simulink model "SolarCar"  (R2025b)
settings: Solver=VariableStepAuto  StartTime=0.0  StopTime=10.0  RelTol=1e-3
undefined symbols (not defined in the file): Line
(part 1 of 2)
settings Model: Creator=nhtyn  LastModifiedBy=nhtyn

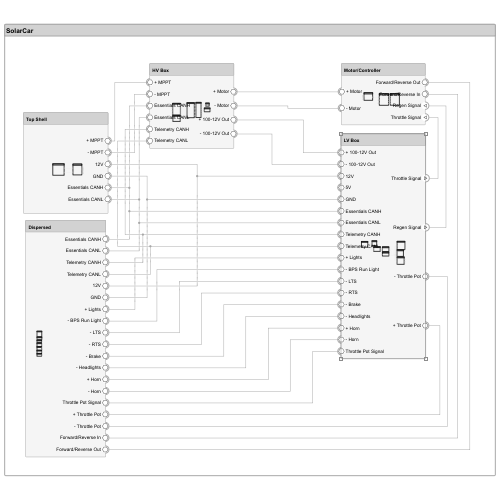
[thumbnail: Simulink's stored preview of the top-level diagram]
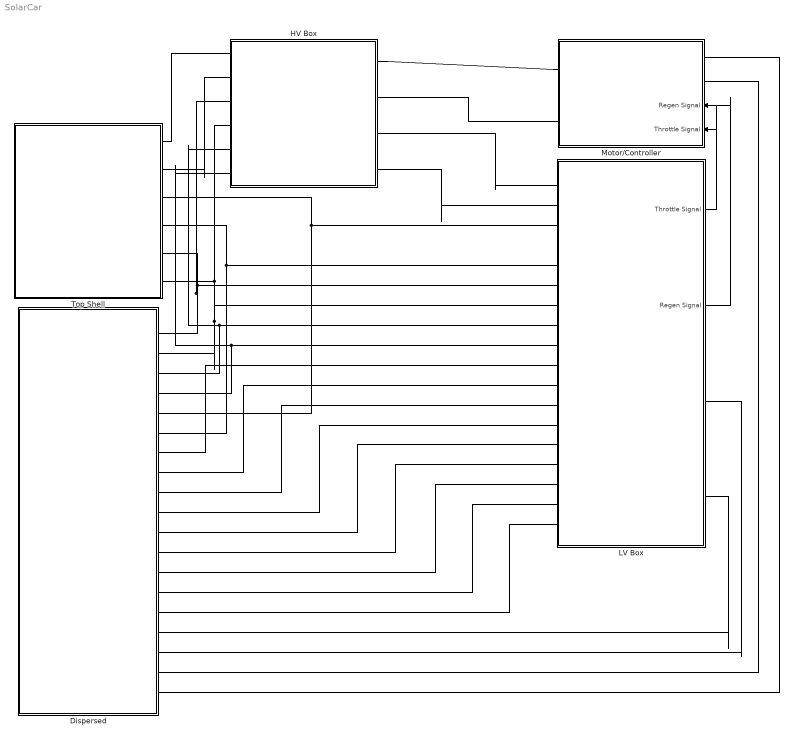
== system SolarCar ==
  Dispersed : Subsystem
      settings: PortSchema="{\"entries\":[{\"content\":{\"headerSize\":26,\"margin\":15,\"minimumSpacing\":25,\"sides\":[{\"content\":{},\"type\":\"ConnectorPlacement.EquallySpacedRectSide\",\"uuid\":\"bc47d88e-4b1b-4064-ab24-769f2538e68d\"},{\"content\":{\"connectorIds\":[\"RConn1\",\"RConn2\",\"RConn3\",\"RConn4\",\"RConn5\",\"RConn6\",\"RConn7\",\"RConn8\",\"RConn9\",\"RConn10\",\"RConn11\",\"RConn12\",\"RConn13\",\"RConn14\",\"RConn15\",\"RConn16\",\"RConn17\",\"RConn18\",\"RConn19\"],\"side\":\"RIGHT\"},\"type\":\"ConnectorPlacement.EquallySpacedRectSide\",\"uuid\":\"fdd62b94-80f2-4d2e-a8f3-223633e3a920\"},{\"content\":{\"side\":\"TOP\"},\"type\":\"ConnectorPlacement.EquallySpacedRectSide\",\"uuid\":\"e8df0b32-bf38-452a-bef9-69ccd7b44596\"}]},\"type\":\"ConnectorPlacement.EquallySpacedConnector\",\"uuid\":\"127e4cb3-ba30-47ff-b0d0-2c5b6f0f1031\"}],\"packageUris\":[\"http://schema.mathworks.com/mf0/Connector/R2020b\"],\"version\":\"1.0\"}"
  HV Box : Subsystem
      settings: PortSchema="{\"entries\":[{\"content\":{\"headerSize\":26,\"margin\":15,\"minimumSpacing\":25,\"sides\":[{\"content\":{\"connectorIds\":[\"RConn5\",\"RConn6\",\"LConn1\",\"LConn2\",\"LConn3\",\"LConn4\"]},\"type\":\"ConnectorPlacement.EquallySpacedRectSide\",\"uuid\":\"c92e0290-dc73-43e5-9f21-68f158b061d1\"},{\"content\":{\"connectorIds\":[\"RConn1\",\"RConn2\",\"RConn3\",\"RConn4\"],\"side\":\"RIGHT\"},\"type\":\"ConnectorPlacement.EquallySpacedRectSide\",\"uuid\":\"be8eb41d-7a66-441b-b503-1306464e1273\"},{\"content\":{\"side\":\"TOP\"},\"type\":\"ConnectorPlacement.EquallySpacedRectSide\",\"uuid\":\"34016d46-a56f-490a-9c85-32531a59f6cc\"}]},\"type\":\"ConnectorPlacement.EquallySpacedConnector\",\"uuid\":\"21576b4b-d4ce-437a-96c9-76a257c64a5e\"}],\"packageUris\":[\"http://schema.mathworks.com/mf0/Connector/R2020b\"],\"version\":\"1.0\"}"
  LV Box : Subsystem
      settings: PortSchema="{\"entries\":[{\"content\":{\"headerSize\":26,\"margin\":15,\"minimumSpacing\":25,\"sides\":[{\"content\":{\"connectorIds\":[\"LConn1\",\"LConn2\",\"LConn3\",\"LConn4\",\"LConn5\",\"LConn6\",\"LConn7\",\"LConn8\",\"LConn9\",\"LConn10\",\"LConn11\",\"LConn12\",\"LConn13\",\"LConn14\",\"LConn15\",\"LConn16\",\"LConn17\",\"LConn18\"]},\"type\":\"ConnectorPlacement.EquallySpacedRectSide\",\"uuid\":\"c92e0290-dc73-43e5-9f21-68f158b061d1\"},{\"content\":{\"connectorIds\":[\"Out1\",\"Out2\",\"RConn2\",\"RConn1\"],\"side\":\"RIGHT\"},\"type\":\"ConnectorPlacement.EquallySpacedRectSide\",\"uuid\":\"be8eb41d-7a66-441b-b503-1306464e1273\"},{\"content\":{\"side\":\"TOP\"},\"type\":\"ConnectorPlacement.EquallySpacedRectSide\",\"uuid\":\"34016d46-a56f-490a-9c85-32531a59f6cc\"}]},\"type\":\"ConnectorPlacement.EquallySpacedConnector\",\"uuid\":\"21576b4b-d4ce-437a-96c9-76a257c64a5e\"}],\"packageUris\":[\"http://schema.mathworks.com/mf0/Connector/R2020b\"],\"version\":\"1.0\"}"
  Motor/Controller : Subsystem
      settings: PortSchema="{\"entries\":[{\"content\":{\"headerSize\":26,\"margin\":15,\"minimumSpacing\":25,\"sides\":[{\"content\":{\"connectorIds\":[\"LConn1\",\"LConn2\"]},\"type\":\"ConnectorPlacement.EquallySpacedRectSide\",\"uuid\":\"c92e0290-dc73-43e5-9f21-68f158b061d1\"},{\"content\":{\"connectorIds\":[\"RConn1\",\"RConn2\",\"In2\",\"In1\"],\"side\":\"RIGHT\"},\"type\":\"ConnectorPlacement.EquallySpacedRectSide\",\"uuid\":\"be8eb41d-7a66-441b-b503-1306464e1273\"},{\"content\":{\"side\":\"TOP\"},\"type\":\"ConnectorPlacement.EquallySpacedRectSide\",\"uuid\":\"34016d46-a56f-490a-9c85-32531a59f6cc\"}]},\"type\":\"ConnectorPlacement.EquallySpacedConnector\",\"uuid\":\"21576b4b-d4ce-437a-96c9-76a257c64a5e\"}],\"packageUris\":[\"http://schema.mathworks.com/mf0/Connector/R2020b\"],\"version\":\"1.0\"}"
  Top Shell : Subsystem
      settings: PortSchema="{\"entries\":[{\"content\":{\"headerSize\":26,\"margin\":15,\"minimumSpacing\":25,\"sides\":[{\"content\":{},\"type\":\"ConnectorPlacement.EquallySpacedRectSide\",\"uuid\":\"c92e0290-dc73-43e5-9f21-68f158b061d1\"},{\"content\":{\"connectorIds\":[\"RConn1\",\"RConn2\",\"RConn3\",\"RConn4\",\"RConn5\",\"RConn6\"],\"side\":\"RIGHT\"},\"type\":\"ConnectorPlacement.EquallySpacedRectSide\",\"uuid\":\"be8eb41d-7a66-441b-b503-1306464e1273\"},{\"content\":{\"side\":\"TOP\"},\"type\":\"ConnectorPlacement.EquallySpacedRectSide\",\"uuid\":\"34016d46-a56f-490a-9c85-32531a59f6cc\"}]},\"type\":\"ConnectorPlacement.EquallySpacedConnector\",\"uuid\":\"21576b4b-d4ce-437a-96c9-76a257c64a5e\"}],\"packageUris\":[\"http://schema.mathworks.com/mf0/Connector/R2020b\"],\"version\":\"1.0\"}"
  wires:
  LV Box/1(Throttle Signal) -> Motor/Controller/1(Throttle Signal)
  LV Box/2(Regen Signal) -> Motor/Controller/2(Regen Signal)
  connections:
  Dispersed/RConn1 -- HV Box/LConn1 -- Top Shell/RConn5 -- LV Box/LConn6
  Top Shell/RConn6 -- HV Box/LConn2 -- Dispersed/RConn2 -- LV Box/LConn7
  HV Box/RConn1 -- Motor/Controller/LConn1
  HV Box/RConn2 -- Motor/Controller/LConn2
  HV Box/RConn5 -- Top Shell/RConn1
  HV Box/RConn6 -- Top Shell/RConn2
  HV Box/RConn3 -- LV Box/LConn1
  HV Box/RConn4 -- LV Box/LConn2
  LV Box/LConn8 -- Dispersed/RConn3 -- HV Box/LConn3
  LV Box/LConn9 -- Dispersed/RConn4 -- HV Box/LConn4
  LV Box/LConn10 -- Dispersed/RConn7
  LV Box/LConn11 -- Dispersed/RConn8
  LV Box/LConn12 -- Dispersed/RConn9
  LV Box/LConn13 -- Dispersed/RConn10
  LV Box/LConn14 -- Dispersed/RConn11
  LV Box/LConn15 -- Dispersed/RConn12
  Dispersed/RConn13 -- LV Box/LConn16
  Dispersed/RConn14 -- LV Box/LConn17
  LV Box/LConn18 -- Dispersed/RConn15
  LV Box/RConn1 -- Dispersed/RConn16
  LV Box/RConn2 -- Dispersed/RConn17
  LV Box/LConn3 -- Top Shell/RConn3 -- Dispersed/RConn5
  LV Box/LConn5 -- Dispersed/RConn6 -- Top Shell/RConn4
  Dispersed/RConn18 -- Motor/Controller/RConn2
  Dispersed/RConn19 -- Motor/Controller/RConn1

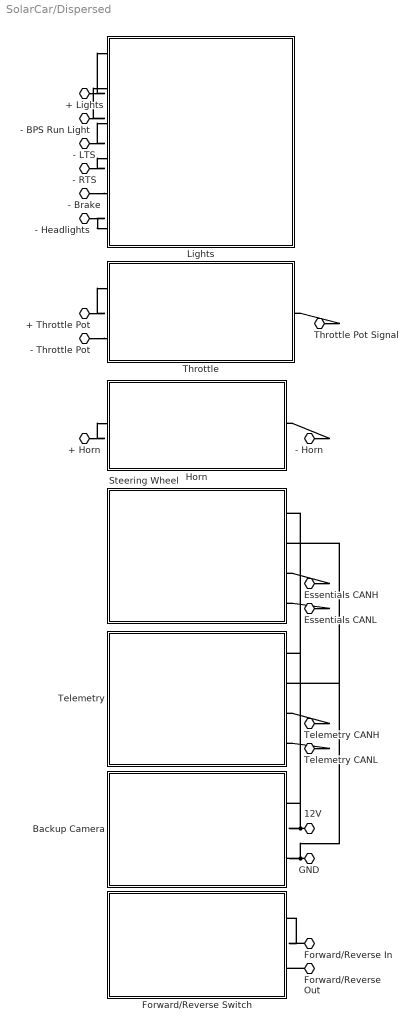
== system SolarCar/Dispersed ==
  Backup Camera : Subsystem
      settings: PortSchema="{\"entries\":[{\"content\":{\"headerSize\":26,\"margin\":15,\"minimumSpacing\":25,\"sides\":[{\"content\":{},\"type\":\"ConnectorPlacement.EquallySpacedRectSide\",\"uuid\":\"16c5a28a-8204-43c6-ae1e-ca56bf00262c\"},{\"content\":{\"connectorIds\":[\"RConn1\",\"RConn2\"],\"side\":\"RIGHT\"},\"type\":\"ConnectorPlacement.EquallySpacedRectSide\",\"uuid\":\"d50f7b79-0d90-4c13-9b04-ddd7ba1c0b17\"},{\"content\":{\"side\":\"TOP\"},\"type\":\"ConnectorPlacement.EquallySpacedRectSide\",\"uuid\":\"232c283e-7372-4332-942a-1b4711a4445f\"}]},\"type\":\"ConnectorPlacement.EquallySpacedConnector\",\"uuid\":\"38533706-c242-4f43-b565-c99062dd3fc1\"}],\"packageUris\":[\"http://schema.mathworks.com/mf0/Connector/R2020b\"],\"version\":\"1.0\"}"
  Forward/Reverse Switch : Subsystem
      settings: PortSchema="{\"entries\":[{\"content\":{\"headerSize\":26,\"margin\":15,\"minimumSpacing\":25,\"sides\":[{\"content\":{},\"type\":\"ConnectorPlacement.EquallySpacedRectSide\",\"uuid\":\"16c5a28a-8204-43c6-ae1e-ca56bf00262c\"},{\"content\":{\"connectorIds\":[\"RConn1\",\"RConn2\"],\"side\":\"RIGHT\"},\"type\":\"ConnectorPlacement.EquallySpacedRectSide\",\"uuid\":\"d50f7b79-0d90-4c13-9b04-ddd7ba1c0b17\"},{\"content\":{\"side\":\"TOP\"},\"type\":\"ConnectorPlacement.EquallySpacedRectSide\",\"uuid\":\"232c283e-7372-4332-942a-1b4711a4445f\"}]},\"type\":\"ConnectorPlacement.EquallySpacedConnector\",\"uuid\":\"38533706-c242-4f43-b565-c99062dd3fc1\"}],\"packageUris\":[\"http://schema.mathworks.com/mf0/Connector/R2020b\"],\"version\":\"1.0\"}"
  Horn : Subsystem
      settings: PortSchema="{\"entries\":[{\"content\":{\"headerSize\":26,\"margin\":15,\"minimumSpacing\":25,\"sides\":[{\"content\":{\"connectorIds\":[\"LConn1\"]},\"type\":\"ConnectorPlacement.EquallySpacedRectSide\",\"uuid\":\"16c5a28a-8204-43c6-ae1e-ca56bf00262c\"},{\"content\":{\"connectorIds\":[\"RConn1\"],\"side\":\"RIGHT\"},\"type\":\"ConnectorPlacement.EquallySpacedRectSide\",\"uuid\":\"d50f7b79-0d90-4c13-9b04-ddd7ba1c0b17\"},{\"content\":{\"side\":\"TOP\"},\"type\":\"ConnectorPlacement.EquallySpacedRectSide\",\"uuid\":\"232c283e-7372-4332-942a-1b4711a4445f\"}]},\"type\":\"ConnectorPlacement.EquallySpacedConnector\",\"uuid\":\"38533706-c242-4f43-b565-c99062dd3fc1\"}],\"packageUris\":[\"http://schema.mathworks.com/mf0/Connector/R2020b\"],\"version\":\"1.0\"}"
  Lights : Subsystem
      settings: PortSchema="{\"entries\":[{\"content\":{\"headerSize\":26,\"margin\":15,\"minimumSpacing\":25,\"sides\":[{\"content\":{\"connectorIds\":[\"LConn1\",\"LConn2\",\"LConn3\",\"LConn4\",\"LConn5\",\"LConn6\"]},\"type\":\"ConnectorPlacement.EquallySpacedRectSide\",\"uuid\":\"16c5a28a-8204-43c6-ae1e-ca56bf00262c\"},{\"content\":{\"side\":\"RIGHT\"},\"type\":\"ConnectorPlacement.EquallySpacedRectSide\",\"uuid\":\"d50f7b79-0d90-4c13-9b04-ddd7ba1c0b17\"},{\"content\":{\"side\":\"TOP\"},\"type\":\"ConnectorPlacement.EquallySpacedRectSide\",\"uuid\":\"232c283e-7372-4332-942a-1b4711a4445f\"}]},\"type\":\"ConnectorPlacement.EquallySpacedConnector\",\"uuid\":\"38533706-c242-4f43-b565-c99062dd3fc1\"}],\"packageUris\":[\"http://schema.mathworks.com/mf0/Connector/R2020b\"],\"version\":\"1.0\"}"
  Steering Wheel : Subsystem
      settings: PortSchema="{\"entries\":[{\"content\":{\"headerSize\":26,\"margin\":15,\"minimumSpacing\":25,\"sides\":[{\"content\":{},\"type\":\"ConnectorPlacement.EquallySpacedRectSide\",\"uuid\":\"bc47d88e-4b1b-4064-ab24-769f2538e68d\"},{\"content\":{\"connectorIds\":[\"RConn1\",\"RConn2\",\"RConn3\",\"RConn4\"],\"side\":\"RIGHT\"},\"type\":\"ConnectorPlacement.EquallySpacedRectSide\",\"uuid\":\"fdd62b94-80f2-4d2e-a8f3-223633e3a920\"},{\"content\":{\"side\":\"TOP\"},\"type\":\"ConnectorPlacement.EquallySpacedRectSide\",\"uuid\":\"e8df0b32-bf38-452a-bef9-69ccd7b44596\"}]},\"type\":\"ConnectorPlacement.EquallySpacedConnector\",\"uuid\":\"127e4cb3-ba30-47ff-b0d0-2c5b6f0f1031\"}],\"packageUris\":[\"http://schema.mathworks.com/mf0/Connector/R2020b\"],\"version\":\"1.0\"}"
  Telemetry : Subsystem
      settings: PortSchema="{\"entries\":[{\"content\":{\"headerSize\":26,\"margin\":15,\"minimumSpacing\":25,\"sides\":[{\"content\":{},\"type\":\"ConnectorPlacement.EquallySpacedRectSide\",\"uuid\":\"bc47d88e-4b1b-4064-ab24-769f2538e68d\"},{\"content\":{\"connectorIds\":[\"RConn1\",\"RConn2\",\"RConn3\",\"RConn4\"],\"side\":\"RIGHT\"},\"type\":\"ConnectorPlacement.EquallySpacedRectSide\",\"uuid\":\"fdd62b94-80f2-4d2e-a8f3-223633e3a920\"},{\"content\":{\"side\":\"TOP\"},\"type\":\"ConnectorPlacement.EquallySpacedRectSide\",\"uuid\":\"e8df0b32-bf38-452a-bef9-69ccd7b44596\"}]},\"type\":\"ConnectorPlacement.EquallySpacedConnector\",\"uuid\":\"127e4cb3-ba30-47ff-b0d0-2c5b6f0f1031\"}],\"packageUris\":[\"http://schema.mathworks.com/mf0/Connector/R2020b\"],\"version\":\"1.0\"}"
  Throttle : Subsystem
      settings: PortSchema="{\"entries\":[{\"content\":{\"headerSize\":26,\"margin\":15,\"minimumSpacing\":25,\"sides\":[{\"content\":{\"connectorIds\":[\"LConn1\",\"LConn2\"]},\"type\":\"ConnectorPlacement.EquallySpacedRectSide\",\"uuid\":\"16c5a28a-8204-43c6-ae1e-ca56bf00262c\"},{\"content\":{\"connectorIds\":[\"RConn1\"],\"side\":\"RIGHT\"},\"type\":\"ConnectorPlacement.EquallySpacedRectSide\",\"uuid\":\"d50f7b79-0d90-4c13-9b04-ddd7ba1c0b17\"},{\"content\":{\"side\":\"TOP\"},\"type\":\"ConnectorPlacement.EquallySpacedRectSide\",\"uuid\":\"232c283e-7372-4332-942a-1b4711a4445f\"}]},\"type\":\"ConnectorPlacement.EquallySpacedConnector\",\"uuid\":\"38533706-c242-4f43-b565-c99062dd3fc1\"}],\"packageUris\":[\"http://schema.mathworks.com/mf0/Connector/R2020b\"],\"version\":\"1.0\"}"
  Essentials CANH : PMIOPort  Side=Right
  Essentials CANL : PMIOPort  Port=2  Side=Right
  Telemetry CANH : PMIOPort  Port=3  Side=Right
  Telemetry CANL : PMIOPort  Port=4  Side=Right
  12V : PMIOPort  Port=5  Side=Right
  GND : PMIOPort  Port=6  Side=Right
  + Lights : PMIOPort  Port=7  Side=Right
  - BPS Run Light : PMIOPort  Port=8  Side=Right
  - LTS : PMIOPort  Port=9  Side=Right
  - RTS : PMIOPort  Port=10  Side=Right
  - Brake : PMIOPort  Port=11  Side=Right
  - Headlights : PMIOPort  Port=12  Side=Right
  + Horn : PMIOPort  Port=13  Side=Right
  - Horn : PMIOPort  Port=14  Side=Right
  Throttle Pot Signal : PMIOPort  Port=15  Side=Right
  + Throttle Pot : PMIOPort  Port=16  Side=Right
  - Throttle Pot : PMIOPort  Port=17  Side=Right
  Forward/Reverse In : PMIOPort  Port=18  Side=Right
  Forward/Reverse Out : PMIOPort  Port=19  Side=Right
  connections:
  Essentials CANH/RConn1 -- Steering Wheel/RConn3
  Essentials CANL/RConn1 -- Steering Wheel/RConn4
  + Lights/RConn1 -- Lights/LConn1
  - BPS Run Light/RConn1 -- Lights/LConn2
  - LTS/RConn1 -- Lights/LConn3
  - RTS/RConn1 -- Lights/LConn4
  - Brake/RConn1 -- Lights/LConn5
  - Headlights/RConn1 -- Lights/LConn6
  + Horn/RConn1 -- Horn/LConn1
  - Horn/RConn1 -- Horn/RConn1
  + Throttle Pot/RConn1 -- Throttle/LConn1
  - Throttle Pot/RConn1 -- Throttle/LConn2
  Throttle Pot Signal/RConn1 -- Throttle/RConn1
  Forward/Reverse In/RConn1 -- Forward/Reverse Switch/RConn1
  Forward/Reverse Out/RConn1 -- Forward/Reverse Switch/RConn2
  12V/RConn1 -- Telemetry/RConn1 -- Steering Wheel/RConn1 -- Backup Camera/RConn1
  GND/RConn1 -- Telemetry/RConn2 -- Steering Wheel/RConn2 -- Backup Camera/RConn2
  Telemetry CANH/RConn1 -- Telemetry/RConn3
  Telemetry CANL/RConn1 -- Telemetry/RConn4

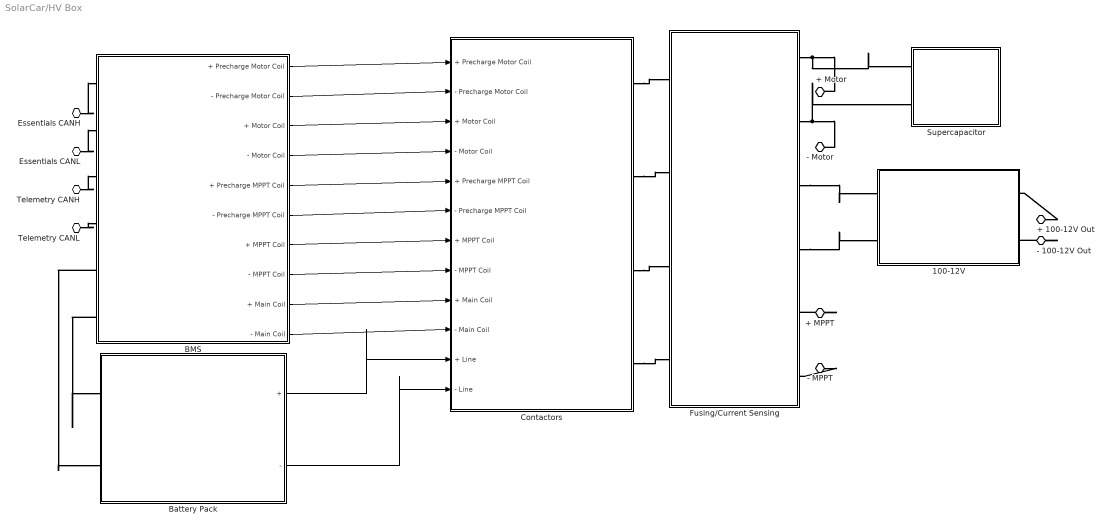
== system SolarCar/HV Box ==
  100-12V : Subsystem
      settings: PortSchema="{\"entries\":[{\"content\":{\"headerSize\":26,\"margin\":15,\"minimumSpacing\":25,\"sides\":[{\"content\":{\"connectorIds\":[\"LConn1\",\"LConn2\"]},\"type\":\"ConnectorPlacement.EquallySpacedRectSide\",\"uuid\":\"c92e0290-dc73-43e5-9f21-68f158b061d1\"},{\"content\":{\"connectorIds\":[\"RConn1\",\"RConn2\"],\"side\":\"RIGHT\"},\"type\":\"ConnectorPlacement.EquallySpacedRectSide\",\"uuid\":\"be8eb41d-7a66-441b-b503-1306464e1273\"},{\"content\":{\"side\":\"TOP\"},\"type\":\"ConnectorPlacement.EquallySpacedRectSide\",\"uuid\":\"34016d46-a56f-490a-9c85-32531a59f6cc\"}]},\"type\":\"ConnectorPlacement.EquallySpacedConnector\",\"uuid\":\"21576b4b-d4ce-437a-96c9-76a257c64a5e\"}],\"packageUris\":[\"http://schema.mathworks.com/mf0/Connector/R2020b\"],\"version\":\"1.0\"}"
  BMS : Subsystem
      settings: PortSchema="{\"entries\":[{\"content\":{\"headerSize\":26,\"margin\":15,\"minimumSpacing\":25,\"sides\":[{\"content\":{\"connectorIds\":[\"LConn1\",\"LConn2\",\"LConn3\",\"LConn4\",\"LConn5\",\"LConn6\"]},\"type\":\"ConnectorPlacement.EquallySpacedRectSide\",\"uuid\":\"c92e0290-dc73-43e5-9f21-68f158b061d1\"},{\"content\":{\"connectorIds\":[\"Out1\",\"Out2\",\"Out3\",\"Out4\",\"Out5\",\"Out6\",\"Out7\",\"Out8\",\"Out9\",\"Out10\"],\"side\":\"RIGHT\"},\"type\":\"ConnectorPlacement.EquallySpacedRectSide\",\"uuid\":\"be8eb41d-7a66-441b-b503-1306464e1273\"},{\"content\":{\"side\":\"TOP\"},\"type\":\"ConnectorPlacement.EquallySpacedRectSide\",\"uuid\":\"34016d46-a56f-490a-9c85-32531a59f6cc\"},{\"content\":{\"side\":\"BOTTOM\"},\"type\":\"ConnectorPlacement.EquallySpacedRectSide\",\"uuid\":\"f63c834d-6003-4ec6-8d44-6b3bc1c3f4f7\"}]},\"type\":\"ConnectorPlacement.EquallySpacedConnector\",\"uuid\":\"21576b4b-d4ce-437a-96c9-76a257c64a5e\"}],\"packageUris\":[\"http://schema.mathworks.com/mf0/Connector/R2020b\"],\"version\":\"1.0\"}"
  Battery Pack : Subsystem
      settings: PortSchema="{\"entries\":[{\"content\":{\"headerSize\":26,\"margin\":15,\"minimumSpacing\":25,\"sides\":[{\"content\":{\"connectorIds\":[\"LConn1\",\"LConn2\"]},\"type\":\"ConnectorPlacement.EquallySpacedRectSide\",\"uuid\":\"c92e0290-dc73-43e5-9f21-68f158b061d1\"},{\"content\":{\"connectorIds\":[\"Out1\",\"Out2\"],\"side\":\"RIGHT\"},\"type\":\"ConnectorPlacement.EquallySpacedRectSide\",\"uuid\":\"be8eb41d-7a66-441b-b503-1306464e1273\"},{\"content\":{\"side\":\"TOP\"},\"type\":\"ConnectorPlacement.EquallySpacedRectSide\",\"uuid\":\"34016d46-a56f-490a-9c85-32531a59f6cc\"}]},\"type\":\"ConnectorPlacement.EquallySpacedConnector\",\"uuid\":\"21576b4b-d4ce-437a-96c9-76a257c64a5e\"}],\"packageUris\":[\"http://schema.mathworks.com/mf0/Connector/R2020b\"],\"version\":\"1.0\"}"
  Contactors : Subsystem
      settings: PortSchema="{\"entries\":[{\"content\":{\"headerSize\":26,\"margin\":15,\"minimumSpacing\":25,\"sides\":[{\"content\":{\"connectorIds\":[\"In1\",\"In2\",\"In3\",\"In4\",\"In5\",\"In6\",\"In7\",\"In8\",\"In9\",\"In10\",\"In11\",\"In12\"]},\"type\":\"ConnectorPlacement.EquallySpacedRectSide\",\"uuid\":\"a524e60d-b40a-408b-8bd2-a27c555355ac\"},{\"content\":{\"connectorIds\":[\"RConn1\",\"RConn3\",\"RConn2\",\"RConn4\"],\"side\":\"RIGHT\"},\"type\":\"ConnectorPlacement.EquallySpacedRectSide\",\"uuid\":\"88e19f78-eac2-4161-9d7e-9c49ae9957fc\"},{\"content\":{\"side\":\"TOP\"},\"type\":\"ConnectorPlacement.EquallySpacedRectSide\",\"uuid\":\"b9255ea4-184a-49ec-9d1c-02386d46c5b2\"}]},\"type\":\"ConnectorPlacement.EquallySpacedConnector\",\"uuid\":\"32913e94-0913-4a3c-90e8-81be48841784\"}],\"packageUris\":[\"http://schema.mathworks.com/mf0/Connector/R2020b\"],\"version\":\"1.0\"}"
  Fusing/Current Sensing : Subsystem
      settings: PortSchema="{\"entries\":[{\"content\":{\"headerSize\":26,\"margin\":15,\"minimumSpacing\":25,\"sides\":[{\"content\":{\"connectorIds\":[\"LConn1\",\"LConn4\",\"LConn2\",\"LConn3\"]},\"type\":\"ConnectorPlacement.EquallySpacedRectSide\",\"uuid\":\"16c5a28a-8204-43c6-ae1e-ca56bf00262c\"},{\"content\":{\"connectorIds\":[\"RConn1\",\"RConn3\",\"RConn2\",\"RConn4\",\"RConn5\",\"RConn6\"],\"side\":\"RIGHT\"},\"type\":\"ConnectorPlacement.EquallySpacedRectSide\",\"uuid\":\"d50f7b79-0d90-4c13-9b04-ddd7ba1c0b17\"},{\"content\":{\"side\":\"TOP\"},\"type\":\"ConnectorPlacement.EquallySpacedRectSide\",\"uuid\":\"232c283e-7372-4332-942a-1b4711a4445f\"}]},\"type\":\"ConnectorPlacement.EquallySpacedConnector\",\"uuid\":\"38533706-c242-4f43-b565-c99062dd3fc1\"}],\"packageUris\":[\"http://schema.mathworks.com/mf0/Connector/R2020b\"],\"version\":\"1.0\"}"
  Supercapacitor : Subsystem
      settings: PortSchema="{\"entries\":[{\"content\":{\"headerSize\":26,\"margin\":15,\"minimumSpacing\":25,\"sides\":[{\"content\":{\"connectorIds\":[\"LConn1\",\"LConn2\"]},\"type\":\"ConnectorPlacement.EquallySpacedRectSide\",\"uuid\":\"7f164fa2-9272-4d7a-9d1b-73fbad559026\"},{\"content\":{\"side\":\"RIGHT\"},\"type\":\"ConnectorPlacement.EquallySpacedRectSide\",\"uuid\":\"4e5c1bb6-197d-43aa-a880-a6796570230e\"},{\"content\":{\"side\":\"TOP\"},\"type\":\"ConnectorPlacement.EquallySpacedRectSide\",\"uuid\":\"a6abaace-1014-4cef-9d43-479b6863617c\"}]},\"type\":\"ConnectorPlacement.EquallySpacedConnector\",\"uuid\":\"97f01c5b-0fe0-4837-90bc-01d73eb3d078\"}],\"packageUris\":[\"http://schema.mathworks.com/mf0/Connector/R2020b\"],\"version\":\"1.0\"}"
  + Motor : PMIOPort  Side=Right
  - Motor : PMIOPort  Port=2  Side=Right
  + 100-12V Out : PMIOPort  Port=3  Side=Right
  - 100-12V Out : PMIOPort  Port=4  Side=Right
  + MPPT : PMIOPort  Port=5  Side=Right
  - MPPT : PMIOPort  Port=6  Side=Right
  Essentials CANH : PMIOPort  Port=7  Side=Left
  Essentials CANL : PMIOPort  Port=8  Side=Left
  Telemetry CANH : PMIOPort  Port=9  Side=Left
  Telemetry CANL : PMIOPort  Port=10  Side=Left
  wires:
  BMS/1(+ Precharge Motor Coil) -> Contactors/1(+ Precharge Motor Coil)
  BMS/2(- Precharge Motor Coil) -> Contactors/2(- Precharge Motor Coil)
  BMS/3(+ Motor Coil) -> Contactors/3(+ Motor Coil)
  Battery Pack/1(+) -> Contactors/11(+ Line)
  Battery Pack/2(-) -> Contactors/12(- Line)
  BMS/4(- Motor Coil) -> Contactors/4(- Motor Coil)
  BMS/5(+ Precharge MPPT Coil) -> Contactors/5(+ Precharge MPPT Coil)
  BMS/6(- Precharge MPPT Coil) -> Contactors/6(- Precharge MPPT Coil)
  BMS/7(+ MPPT Coil) -> Contactors/7(+ MPPT Coil)
  BMS/8(- MPPT Coil) -> Contactors/8(- MPPT Coil)
  BMS/9(+ Main Coil) -> Contactors/9(+ Main Coil)
  BMS/10(- Main Coil) -> Contactors/10(- Main Coil)
  connections:
  Contactors/RConn4 -- Fusing/Current Sensing/LConn3
  Contactors/RConn3 -- Fusing/Current Sensing/LConn4
  Contactors/RConn1 -- Fusing/Current Sensing/LConn1
  Contactors/RConn2 -- Fusing/Current Sensing/LConn2
  Fusing/Current Sensing/RConn2 -- 100-12V/LConn1
  Fusing/Current Sensing/RConn4 -- 100-12V/LConn2
  Fusing/Current Sensing/RConn1 -- Supercapacitor/LConn1 -- + Motor/RConn1
  Fusing/Current Sensing/RConn3 -- Supercapacitor/LConn2 -- - Motor/RConn1
  - MPPT/RConn1 -- Fusing/Current Sensing/RConn6
  + MPPT/RConn1 -- Fusing/Current Sensing/RConn5
  + 100-12V Out/RConn1 -- 100-12V/RConn1
  - 100-12V Out/RConn1 -- 100-12V/RConn2
  Essentials CANH/RConn1 -- BMS/LConn1
  Essentials CANL/RConn1 -- BMS/LConn2
  Telemetry CANH/RConn1 -- BMS/LConn3
  Telemetry CANL/RConn1 -- BMS/LConn4
  BMS/LConn5 -- Battery Pack/LConn2
  BMS/LConn6 -- Battery Pack/LConn1

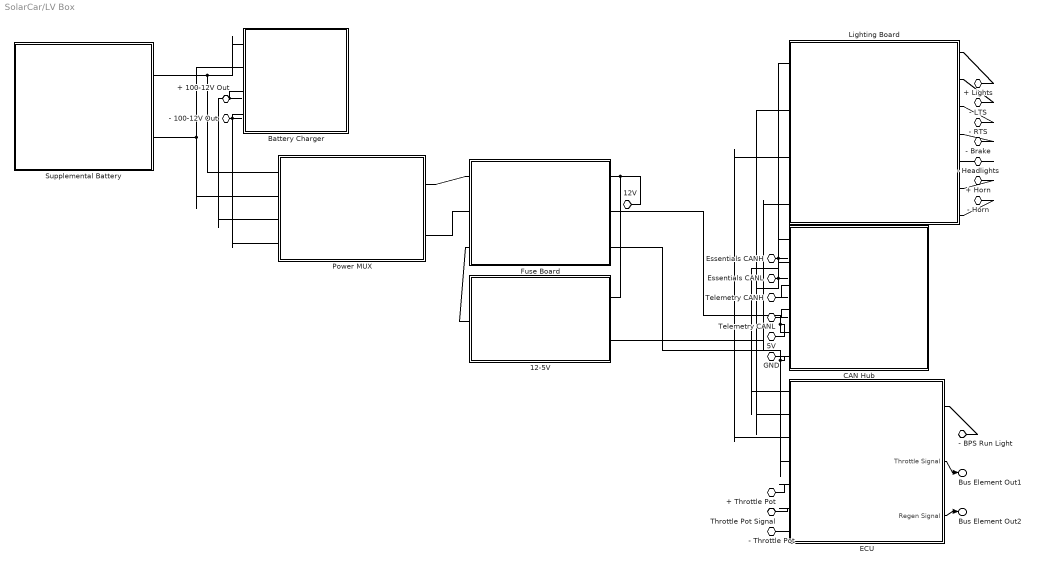
== system SolarCar/LV Box ==
  12-5V : Subsystem
      settings: PortSchema="{\"entries\":[{\"content\":{\"headerSize\":26,\"margin\":15,\"minimumSpacing\":25,\"sides\":[{\"content\":{\"connectorIds\":[\"RConn1\"]},\"type\":\"ConnectorPlacement.EquallySpacedRectSide\",\"uuid\":\"e398aa85-cf01-454b-8c65-40a3b68188cb\"},{\"content\":{\"connectorIds\":[\"LConn1\",\"LConn2\"],\"side\":\"RIGHT\"},\"type\":\"ConnectorPlacement.EquallySpacedRectSide\",\"uuid\":\"9e40fc98-7fa4-4457-a2a2-72d8b3bd46fd\"},{\"content\":{\"side\":\"TOP\"},\"type\":\"ConnectorPlacement.EquallySpacedRectSide\",\"uuid\":\"c0cef17d-c612-441a-9462-c940c3f96980\"}]},\"type\":\"ConnectorPlacement.EquallySpacedConnector\",\"uuid\":\"0ce439f7-0020-43e2-bdb3-8e0f3c386e01\"}],\"packageUris\":[\"http://schema.mathworks.com/mf0/Connector/R2020b\"],\"version\":\"1.0\"}"
  Battery Charger : Subsystem
      settings: PortSchema="{\"entries\":[{\"content\":{\"headerSize\":26,\"margin\":15,\"minimumSpacing\":25,\"sides\":[{\"content\":{\"connectorIds\":[\"LConn1\",\"LConn2\",\"RConn1\",\"RConn2\"]},\"type\":\"ConnectorPlacement.EquallySpacedRectSide\",\"uuid\":\"7f164fa2-9272-4d7a-9d1b-73fbad559026\"},{\"content\":{\"side\":\"RIGHT\"},\"type\":\"ConnectorPlacement.EquallySpacedRectSide\",\"uuid\":\"4e5c1bb6-197d-43aa-a880-a6796570230e\"},{\"content\":{\"side\":\"TOP\"},\"type\":\"ConnectorPlacement.EquallySpacedRectSide\",\"uuid\":\"a6abaace-1014-4cef-9d43-479b6863617c\"}]},\"type\":\"ConnectorPlacement.EquallySpacedConnector\",\"uuid\":\"97f01c5b-0fe0-4837-90bc-01d73eb3d078\"}],\"packageUris\":[\"http://schema.mathworks.com/mf0/Connector/R2020b\"],\"version\":\"1.0\"}"
  CAN Hub : Subsystem
      settings: PortSchema="{\"entries\":[{\"content\":{\"headerSize\":26,\"margin\":15,\"minimumSpacing\":25,\"sides\":[{\"content\":{\"connectorIds\":[\"LConn1\",\"LConn2\",\"LConn3\",\"LConn4\",\"LConn5\",\"LConn6\"]},\"type\":\"ConnectorPlacement.EquallySpacedRectSide\",\"uuid\":\"16c5a28a-8204-43c6-ae1e-ca56bf00262c\"},{\"content\":{\"side\":\"RIGHT\"},\"type\":\"ConnectorPlacement.EquallySpacedRectSide\",\"uuid\":\"d50f7b79-0d90-4c13-9b04-ddd7ba1c0b17\"},{\"content\":{\"side\":\"TOP\"},\"type\":\"ConnectorPlacement.EquallySpacedRectSide\",\"uuid\":\"232c283e-7372-4332-942a-1b4711a4445f\"}]},\"type\":\"ConnectorPlacement.EquallySpacedConnector\",\"uuid\":\"38533706-c242-4f43-b565-c99062dd3fc1\"}],\"packageUris\":[\"http://schema.mathworks.com/mf0/Connector/R2020b\"],\"version\":\"1.0\"}"
  ECU : Subsystem
      settings: PortSchema="{\"entries\":[{\"content\":{\"headerSize\":26,\"margin\":15,\"minimumSpacing\":25,\"sides\":[{\"content\":{\"connectorIds\":[\"LConn1\",\"LConn2\",\"LConn3\",\"LConn4\",\"LConn5\",\"LConn6\",\"LConn7\"]},\"type\":\"ConnectorPlacement.EquallySpacedRectSide\",\"uuid\":\"c92e0290-dc73-43e5-9f21-68f158b061d1\"},{\"content\":{\"connectorIds\":[\"RConn1\",\"Out1\",\"Out2\"],\"side\":\"RIGHT\"},\"type\":\"ConnectorPlacement.EquallySpacedRectSide\",\"uuid\":\"be8eb41d-7a66-441b-b503-1306464e1273\"},{\"content\":{\"side\":\"TOP\"},\"type\":\"ConnectorPlacement.EquallySpacedRectSide\",\"uuid\":\"34016d46-a56f-490a-9c85-32531a59f6cc\"}]},\"type\":\"ConnectorPlacement.EquallySpacedConnector\",\"uuid\":\"21576b4b-d4ce-437a-96c9-76a257c64a5e\"}],\"packageUris\":[\"http://schema.mathworks.com/mf0/Connector/R2020b\"],\"version\":\"1.0\"}"
  Fuse Board : Subsystem
      settings: PortSchema="{\"entries\":[{\"content\":{\"headerSize\":26,\"margin\":15,\"minimumSpacing\":25,\"sides\":[{\"content\":{\"connectorIds\":[\"LConn1\",\"LConn2\",\"LConn3\"]},\"type\":\"ConnectorPlacement.EquallySpacedRectSide\",\"uuid\":\"c92e0290-dc73-43e5-9f21-68f158b061d1\"},{\"content\":{\"connectorIds\":[\"RConn1\",\"RConn2\",\"RConn3\"],\"side\":\"RIGHT\"},\"type\":\"ConnectorPlacement.EquallySpacedRectSide\",\"uuid\":\"be8eb41d-7a66-441b-b503-1306464e1273\"},{\"content\":{\"side\":\"TOP\"},\"type\":\"ConnectorPlacement.EquallySpacedRectSide\",\"uuid\":\"34016d46-a56f-490a-9c85-32531a59f6cc\"}]},\"type\":\"ConnectorPlacement.EquallySpacedConnector\",\"uuid\":\"21576b4b-d4ce-437a-96c9-76a257c64a5e\"}],\"packageUris\":[\"http://schema.mathworks.com/mf0/Connector/R2020b\"],\"version\":\"1.0\"}"
  Lighting Board : Subsystem
      settings: PortSchema="{\"entries\":[{\"content\":{\"headerSize\":26,\"margin\":15,\"minimumSpacing\":25,\"sides\":[{\"content\":{\"connectorIds\":[\"LConn1\",\"LConn2\",\"LConn3\",\"LConn4\"]},\"type\":\"ConnectorPlacement.EquallySpacedRectSide\",\"uuid\":\"c92e0290-dc73-43e5-9f21-68f158b061d1\"},{\"content\":{\"connectorIds\":[\"RConn2\",\"RConn3\",\"RConn1\",\"RConn4\",\"RConn5\",\"RConn6\",\"RConn7\"],\"side\":\"RIGHT\"},\"type\":\"ConnectorPlacement.EquallySpacedRectSide\",\"uuid\":\"be8eb41d-7a66-441b-b503-1306464e1273\"},{\"content\":{\"side\":\"TOP\"},\"type\":\"ConnectorPlacement.EquallySpacedRectSide\",\"uuid\":\"34016d46-a56f-490a-9c85-32531a59f6cc\"},{\"content\":{\"side\":\"BOTTOM\"},\"type\":\"ConnectorPlacement.EquallySpacedRectSide\",\"uuid\":\"089da668-218a-4509-a90e-e522bf51239f\"}]},\"type\":\"ConnectorPlacement.EquallySpacedConnector\",\"uuid\":\"21576b4b-d4ce-437a-96c9-76a257c64a5e\"}],\"packageUris\":[\"http://schema.mathworks.com/mf0/Connector/R2020b\"],\"version\":\"1.0\"}"
  Power MUX : Subsystem
      settings: PortSchema="{\"entries\":[{\"content\":{\"headerSize\":26,\"margin\":15,\"minimumSpacing\":25,\"sides\":[{\"content\":{\"connectorIds\":[\"LConn1\",\"LConn2\",\"LConn3\",\"RConn3\"]},\"type\":\"ConnectorPlacement.EquallySpacedRectSide\",\"uuid\":\"c92e0290-dc73-43e5-9f21-68f158b061d1\"},{\"content\":{\"connectorIds\":[\"RConn1\",\"RConn2\"],\"side\":\"RIGHT\"},\"type\":\"ConnectorPlacement.EquallySpacedRectSide\",\"uuid\":\"be8eb41d-7a66-441b-b503-1306464e1273\"},{\"content\":{\"side\":\"TOP\"},\"type\":\"ConnectorPlacement.EquallySpacedRectSide\",\"uuid\":\"34016d46-a56f-490a-9c85-32531a59f6cc\"},{\"content\":{\"side\":\"BOTTOM\"},\"type\":\"ConnectorPlacement.EquallySpacedRectSide\",\"uuid\":\"c5320d22-5298-4b0f-919e-298988f1412c\"}]},\"type\":\"ConnectorPlacement.EquallySpacedConnector\",\"uuid\":\"21576b4b-d4ce-437a-96c9-76a257c64a5e\"}],\"packageUris\":[\"http://schema.mathworks.com/mf0/Connector/R2020b\"],\"version\":\"1.0\"}"
  Supplemental Battery : Subsystem
      settings: PortSchema="{\"entries\":[{\"content\":{\"headerSize\":26,\"margin\":15,\"minimumSpacing\":25,\"sides\":[{\"content\":{},\"type\":\"ConnectorPlacement.EquallySpacedRectSide\",\"uuid\":\"c92e0290-dc73-43e5-9f21-68f158b061d1\"},{\"content\":{\"connectorIds\":[\"RConn1\",\"RConn2\"],\"side\":\"RIGHT\"},\"type\":\"ConnectorPlacement.EquallySpacedRectSide\",\"uuid\":\"be8eb41d-7a66-441b-b503-1306464e1273\"},{\"content\":{\"side\":\"TOP\"},\"type\":\"ConnectorPlacement.EquallySpacedRectSide\",\"uuid\":\"34016d46-a56f-490a-9c85-32531a59f6cc\"}]},\"type\":\"ConnectorPlacement.EquallySpacedConnector\",\"uuid\":\"21576b4b-d4ce-437a-96c9-76a257c64a5e\"}],\"packageUris\":[\"http://schema.mathworks.com/mf0/Connector/R2020b\"],\"version\":\"1.0\"}"
  + 100-12V Out : PMIOPort  Side=Left
  - 100-12V Out : PMIOPort  Port=2  Side=Left
  12V : PMIOPort  Port=3  Side=Left
  5V : PMIOPort  Port=4  Side=Left
  GND : PMIOPort  Port=5  Side=Left
  Essentials CANH : PMIOPort  Port=6  Side=Left
  Essentials CANL : PMIOPort  Port=7  Side=Left
  Telemetry CANH : PMIOPort  Port=8  Side=Left
  Telemetry CANL : PMIOPort  Port=9  Side=Left
  + Lights : PMIOPort  Port=10  Side=Left
  - BPS Run Light : PMIOPort  Port=11  Side=Left
  - LTS : PMIOPort  Port=12  Side=Left
  - RTS : PMIOPort  Port=13  Side=Left
  - Brake : PMIOPort  Port=14  Side=Left
  - Headlights : PMIOPort  Port=15  Side=Left
  + Horn : PMIOPort  Port=16  Side=Left
  - Horn : PMIOPort  Port=17  Side=Left
  + Throttle Pot : PMIOPort  Port=18  Side=Right
  - Throttle Pot : PMIOPort  Port=19  Side=Right
  Throttle Pot Signal : PMIOPort  Port=20  Side=Left
  Bus Element Out1 : Outport  PortName=Throttle Signal
  Bus Element Out2 : Outport  Port=2  PortName=Regen Signal
  wires:
  ECU/1(Throttle Signal) -> Bus Element Out1/1
  ECU/2(Regen Signal) -> Bus Element Out2/1
  connections:
  Essentials CANH/RConn1 -- CAN Hub/LConn1 -- Lighting Board/LConn1 -- ECU/LConn1
  Essentials CANL/RConn1 -- CAN Hub/LConn2 -- Lighting Board/LConn2 -- ECU/LConn2
  + Lights/RConn1 -- Lighting Board/RConn2
  - LTS/RConn1 -- Lighting Board/RConn3
  - RTS/RConn1 -- Lighting Board/RConn1
  - Brake/RConn1 -- Lighting Board/RConn4
  - Headlights/RConn1 -- Lighting Board/RConn5
  Telemetry CANH/RConn1 -- CAN Hub/LConn3
  Telemetry CANL/RConn1 -- CAN Hub/LConn4
  Supplemental Battery/RConn1 -- Battery Charger/LConn1 -- Power MUX/LConn1
  Supplemental Battery/RConn2 -- Battery Charger/LConn2 -- Power MUX/LConn2
  + 100-12V Out/RConn1 -- Battery Charger/RConn1 -- Power MUX/LConn3
  - 100-12V Out/RConn1 -- Battery Charger/RConn2 -- Power MUX/RConn3
  Power MUX/RConn1 -- Fuse Board/LConn1
  Power MUX/RConn2 -- Fuse Board/LConn2
  ECU/LConn5 -- + Throttle Pot/RConn1
  ECU/LConn7 -- - Throttle Pot/RConn1
  ECU/LConn6 -- Throttle Pot Signal/RConn1
  + Horn/RConn1 -- Lighting Board/RConn6
  - Horn/RConn1 -- Lighting Board/RConn7
  - BPS Run Light/RConn1 -- ECU/RConn1
  Fuse Board/RConn3 -- CAN Hub/LConn6 -- ECU/LConn4 -- 12-5V/LConn2 -- Lighting Board/LConn4 -- GND/RConn1
  Fuse Board/RConn1 -- 12V/RConn1 -- 12-5V/LConn1
  12-5V/RConn1 -- Fuse Board/LConn3
  Fuse Board/RConn2 -- ECU/LConn3 -- CAN Hub/LConn5 -- Lighting Board/LConn3 -- 5V/RConn1

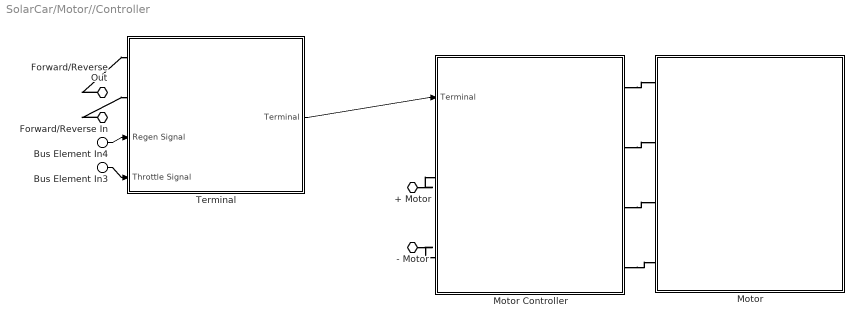
== system SolarCar/Motor//Controller ==
  Bus Element In3 : Inport  PortName=Throttle Signal
  Bus Element In4 : Inport  Port=2  PortName=Regen Signal
  Motor : Subsystem
      settings: PortSchema="{\"entries\":[{\"content\":{\"headerSize\":26,\"margin\":15,\"minimumSpacing\":25,\"sides\":[{\"content\":{\"connectorIds\":[\"LConn1\",\"LConn2\",\"LConn3\",\"LConn4\"]},\"type\":\"ConnectorPlacement.EquallySpacedRectSide\",\"uuid\":\"c92e0290-dc73-43e5-9f21-68f158b061d1\"},{\"content\":{\"side\":\"RIGHT\"},\"type\":\"ConnectorPlacement.EquallySpacedRectSide\",\"uuid\":\"be8eb41d-7a66-441b-b503-1306464e1273\"},{\"content\":{\"side\":\"TOP\"},\"type\":\"ConnectorPlacement.EquallySpacedRectSide\",\"uuid\":\"34016d46-a56f-490a-9c85-32531a59f6cc\"}]},\"type\":\"ConnectorPlacement.EquallySpacedConnector\",\"uuid\":\"21576b4b-d4ce-437a-96c9-76a257c64a5e\"}],\"packageUris\":[\"http://schema.mathworks.com/mf0/Connector/R2020b\"],\"version\":\"1.0\"}"
  Motor Controller : Subsystem
      settings: PortSchema="{\"entries\":[{\"content\":{\"headerSize\":26,\"margin\":15,\"minimumSpacing\":25,\"sides\":[{\"content\":{\"connectorIds\":[\"In1\",\"LConn1\",\"LConn2\"]},\"type\":\"ConnectorPlacement.EquallySpacedRectSide\",\"uuid\":\"c92e0290-dc73-43e5-9f21-68f158b061d1\"},{\"content\":{\"connectorIds\":[\"RConn1\",\"RConn2\",\"RConn3\",\"RConn4\"],\"side\":\"RIGHT\"},\"type\":\"ConnectorPlacement.EquallySpacedRectSide\",\"uuid\":\"be8eb41d-7a66-441b-b503-1306464e1273\"},{\"content\":{\"side\":\"TOP\"},\"type\":\"ConnectorPlacement.EquallySpacedRectSide\",\"uuid\":\"34016d46-a56f-490a-9c85-32531a59f6cc\"}]},\"type\":\"ConnectorPlacement.EquallySpacedConnector\",\"uuid\":\"21576b4b-d4ce-437a-96c9-76a257c64a5e\"}],\"packageUris\":[\"http://schema.mathworks.com/mf0/Connector/R2020b\"],\"version\":\"1.0\"}"
  Terminal : Subsystem
      settings: PortSchema="{\"entries\":[{\"content\":{\"headerSize\":26,\"margin\":15,\"minimumSpacing\":25,\"sides\":[{\"content\":{\"connectorIds\":[\"LConn1\",\"LConn2\",\"In1\",\"In2\"]},\"type\":\"ConnectorPlacement.EquallySpacedRectSide\",\"uuid\":\"16c5a28a-8204-43c6-ae1e-ca56bf00262c\"},{\"content\":{\"connectorIds\":[\"Out1\"],\"side\":\"RIGHT\"},\"type\":\"ConnectorPlacement.EquallySpacedRectSide\",\"uuid\":\"d50f7b79-0d90-4c13-9b04-ddd7ba1c0b17\"},{\"content\":{\"side\":\"TOP\"},\"type\":\"ConnectorPlacement.EquallySpacedRectSide\",\"uuid\":\"232c283e-7372-4332-942a-1b4711a4445f\"}]},\"type\":\"ConnectorPlacement.EquallySpacedConnector\",\"uuid\":\"38533706-c242-4f43-b565-c99062dd3fc1\"}],\"packageUris\":[\"http://schema.mathworks.com/mf0/Connector/R2020b\"],\"version\":\"1.0\"}"
  + Motor : PMIOPort  Side=Left
  - Motor : PMIOPort  Port=2  Side=Left
  Forward/Reverse Out : PMIOPort  Port=3  Side=Right
  Forward/Reverse In : PMIOPort  Port=4  Side=Right
  wires:
  Terminal/1(Terminal) -> Motor Controller/1(Terminal)
  Bus Element In4/1 -> Terminal/1(Regen Signal)
  Bus Element In3/1 -> Terminal/2(Throttle Signal)
  connections:
  + Motor/RConn1 -- Motor Controller/LConn1
  Motor Controller/RConn1 -- Motor/LConn1
  Motor Controller/RConn2 -- Motor/LConn2
  Motor Controller/RConn3 -- Motor/LConn3
  Motor Controller/RConn4 -- Motor/LConn4
  Forward/Reverse Out/RConn1 -- Terminal/LConn1
  Forward/Reverse In/RConn1 -- Terminal/LConn2
  - Motor/RConn1 -- Motor Controller/LConn2

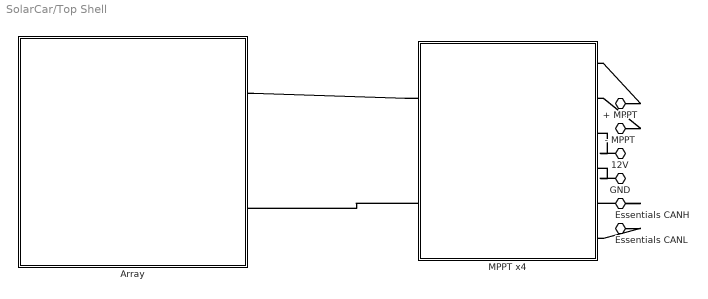
== system SolarCar/Top Shell ==
  Array : Subsystem
      settings: PortSchema="{\"entries\":[{\"content\":{\"headerSize\":26,\"margin\":15,\"minimumSpacing\":25,\"sides\":[{\"content\":{},\"type\":\"ConnectorPlacement.EquallySpacedRectSide\",\"uuid\":\"e398aa85-cf01-454b-8c65-40a3b68188cb\"},{\"content\":{\"connectorIds\":[\"RConn1\",\"RConn2\"],\"side\":\"RIGHT\"},\"type\":\"ConnectorPlacement.EquallySpacedRectSide\",\"uuid\":\"9e40fc98-7fa4-4457-a2a2-72d8b3bd46fd\"},{\"content\":{\"side\":\"TOP\"},\"type\":\"ConnectorPlacement.EquallySpacedRectSide\",\"uuid\":\"c0cef17d-c612-441a-9462-c940c3f96980\"}]},\"type\":\"ConnectorPlacement.EquallySpacedConnector\",\"uuid\":\"0ce439f7-0020-43e2-bdb3-8e0f3c386e01\"}],\"packageUris\":[\"http://schema.mathworks.com/mf0/Connector/R2020b\"],\"version\":\"1.0\"}"
  MPPT x4 : Subsystem
      settings: PortSchema="{\"entries\":[{\"content\":{\"headerSize\":26,\"margin\":15,\"minimumSpacing\":25,\"sides\":[{\"content\":{\"connectorIds\":[\"LConn1\",\"LConn2\"]},\"type\":\"ConnectorPlacement.EquallySpacedRectSide\",\"uuid\":\"e398aa85-cf01-454b-8c65-40a3b68188cb\"},{\"content\":{\"connectorIds\":[\"RConn1\",\"RConn2\",\"RConn3\",\"RConn4\",\"RConn5\",\"RConn6\"],\"side\":\"RIGHT\"},\"type\":\"ConnectorPlacement.EquallySpacedRectSide\",\"uuid\":\"9e40fc98-7fa4-4457-a2a2-72d8b3bd46fd\"},{\"content\":{\"side\":\"TOP\"},\"type\":\"ConnectorPlacement.EquallySpacedRectSide\",\"uuid\":\"c0cef17d-c612-441a-9462-c940c3f96980\"}]},\"type\":\"ConnectorPlacement.EquallySpacedConnector\",\"uuid\":\"0ce439f7-0020-43e2-bdb3-8e0f3c386e01\"}],\"packageUris\":[\"http://schema.mathworks.com/mf0/Connector/R2020b\"],\"version\":\"1.0\"}"
  + MPPT : PMIOPort  Side=Right
  - MPPT : PMIOPort  Port=2  Side=Right
  12V : PMIOPort  Port=3  Side=Right
  GND : PMIOPort  Port=4  Side=Right
  Essentials CANH : PMIOPort  Port=5  Side=Right
  Essentials CANL : PMIOPort  Port=6  Side=Right
  connections:
  Essentials CANH/RConn1 -- MPPT x4/RConn5
  Essentials CANL/RConn1 -- MPPT x4/RConn6
  + MPPT/RConn1 -- MPPT x4/RConn1
  - MPPT/RConn1 -- MPPT x4/RConn2
  MPPT x4/LConn1 -- Array/RConn1
  MPPT x4/LConn2 -- Array/RConn2
  GND/RConn1 -- MPPT x4/RConn4
  12V/RConn1 -- MPPT x4/RConn3

== system SolarCar/Dispersed/Backup Camera ==
  12V : PMIOPort  Side=Right
  GND : PMIOPort  Port=2  Side=Right

== system SolarCar/Dispersed/Forward//Reverse Switch ==
  Forward/Reverse In : PMIOPort  Side=Right
  Forward/Reverse Out : PMIOPort  Port=2  Side=Right

== system SolarCar/Dispersed/Horn ==
  + Horn : PMIOPort  Side=Left
  - Horn : PMIOPort  Port=2  Side=Right

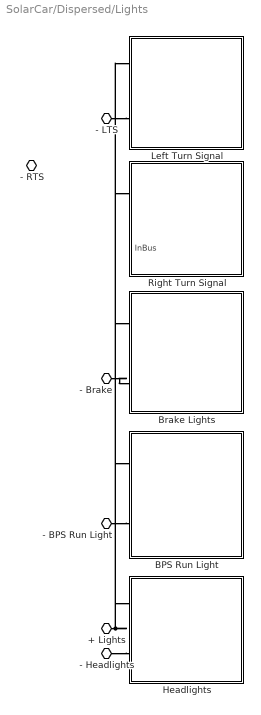
== system SolarCar/Dispersed/Lights ==
  BPS Run Light : Subsystem
      settings: PortSchema="{\"entries\":[{\"content\":{\"headerSize\":26,\"margin\":15,\"minimumSpacing\":25,\"sides\":[{\"content\":{\"connectorIds\":[\"LConn1\",\"LConn2\"]},\"type\":\"ConnectorPlacement.EquallySpacedRectSide\",\"uuid\":\"16c5a28a-8204-43c6-ae1e-ca56bf00262c\"},{\"content\":{\"side\":\"RIGHT\"},\"type\":\"ConnectorPlacement.EquallySpacedRectSide\",\"uuid\":\"d50f7b79-0d90-4c13-9b04-ddd7ba1c0b17\"},{\"content\":{\"side\":\"TOP\"},\"type\":\"ConnectorPlacement.EquallySpacedRectSide\",\"uuid\":\"232c283e-7372-4332-942a-1b4711a4445f\"}]},\"type\":\"ConnectorPlacement.EquallySpacedConnector\",\"uuid\":\"38533706-c242-4f43-b565-c99062dd3fc1\"}],\"packageUris\":[\"http://schema.mathworks.com/mf0/Connector/R2020b\"],\"version\":\"1.0\"}"
  Brake Lights : Subsystem
      settings: PortSchema="{\"entries\":[{\"content\":{\"headerSize\":26,\"margin\":15,\"minimumSpacing\":25,\"sides\":[{\"content\":{\"connectorIds\":[\"LConn1\",\"LConn2\"]},\"type\":\"ConnectorPlacement.EquallySpacedRectSide\",\"uuid\":\"16c5a28a-8204-43c6-ae1e-ca56bf00262c\"},{\"content\":{\"side\":\"RIGHT\"},\"type\":\"ConnectorPlacement.EquallySpacedRectSide\",\"uuid\":\"d50f7b79-0d90-4c13-9b04-ddd7ba1c0b17\"},{\"content\":{\"side\":\"TOP\"},\"type\":\"ConnectorPlacement.EquallySpacedRectSide\",\"uuid\":\"232c283e-7372-4332-942a-1b4711a4445f\"}]},\"type\":\"ConnectorPlacement.EquallySpacedConnector\",\"uuid\":\"38533706-c242-4f43-b565-c99062dd3fc1\"}],\"packageUris\":[\"http://schema.mathworks.com/mf0/Connector/R2020b\"],\"version\":\"1.0\"}"
  Headlights : Subsystem
      settings: PortSchema="{\"entries\":[{\"content\":{\"headerSize\":26,\"margin\":15,\"minimumSpacing\":25,\"sides\":[{\"content\":{\"connectorIds\":[\"LConn1\",\"LConn2\"]},\"type\":\"ConnectorPlacement.EquallySpacedRectSide\",\"uuid\":\"16c5a28a-8204-43c6-ae1e-ca56bf00262c\"},{\"content\":{\"side\":\"RIGHT\"},\"type\":\"ConnectorPlacement.EquallySpacedRectSide\",\"uuid\":\"d50f7b79-0d90-4c13-9b04-ddd7ba1c0b17\"},{\"content\":{\"side\":\"TOP\"},\"type\":\"ConnectorPlacement.EquallySpacedRectSide\",\"uuid\":\"232c283e-7372-4332-942a-1b4711a4445f\"}]},\"type\":\"ConnectorPlacement.EquallySpacedConnector\",\"uuid\":\"38533706-c242-4f43-b565-c99062dd3fc1\"}],\"packageUris\":[\"http://schema.mathworks.com/mf0/Connector/R2020b\"],\"version\":\"1.0\"}"
  Left Turn Signal : Subsystem
      settings: PortSchema="{\"entries\":[{\"content\":{\"headerSize\":26,\"margin\":15,\"minimumSpacing\":25,\"sides\":[{\"content\":{\"connectorIds\":[\"LConn1\",\"LConn2\"]},\"type\":\"ConnectorPlacement.EquallySpacedRectSide\",\"uuid\":\"16c5a28a-8204-43c6-ae1e-ca56bf00262c\"},{\"content\":{\"side\":\"RIGHT\"},\"type\":\"ConnectorPlacement.EquallySpacedRectSide\",\"uuid\":\"d50f7b79-0d90-4c13-9b04-ddd7ba1c0b17\"},{\"content\":{\"side\":\"TOP\"},\"type\":\"ConnectorPlacement.EquallySpacedRectSide\",\"uuid\":\"232c283e-7372-4332-942a-1b4711a4445f\"}]},\"type\":\"ConnectorPlacement.EquallySpacedConnector\",\"uuid\":\"38533706-c242-4f43-b565-c99062dd3fc1\"}],\"packageUris\":[\"http://schema.mathworks.com/mf0/Connector/R2020b\"],\"version\":\"1.0\"}"
  Right Turn Signal : Subsystem
      settings: PortSchema="{\"entries\":[{\"content\":{\"headerSize\":26,\"margin\":15,\"minimumSpacing\":25,\"sides\":[{\"content\":{\"connectorIds\":[\"LConn1\",\"In1\"]},\"type\":\"ConnectorPlacement.EquallySpacedRectSide\",\"uuid\":\"16c5a28a-8204-43c6-ae1e-ca56bf00262c\"},{\"content\":{\"side\":\"RIGHT\"},\"type\":\"ConnectorPlacement.EquallySpacedRectSide\",\"uuid\":\"d50f7b79-0d90-4c13-9b04-ddd7ba1c0b17\"},{\"content\":{\"side\":\"TOP\"},\"type\":\"ConnectorPlacement.EquallySpacedRectSide\",\"uuid\":\"232c283e-7372-4332-942a-1b4711a4445f\"}]},\"type\":\"ConnectorPlacement.EquallySpacedConnector\",\"uuid\":\"38533706-c242-4f43-b565-c99062dd3fc1\"}],\"packageUris\":[\"http://schema.mathworks.com/mf0/Connector/R2020b\"],\"version\":\"1.0\"}"
  + Lights : PMIOPort  Side=Left
  - BPS Run Light : PMIOPort  Port=2  Side=Left
  - LTS : PMIOPort  Port=3  Side=Left
  - RTS : PMIOPort  Port=4  Side=Left
  - Brake : PMIOPort  Port=5  Side=Left
  - Headlights : PMIOPort  Port=6  Side=Left
  wires:
  ? -> Right Turn Signal/1(InBus)
  connections:
  + Lights/RConn1 -- Right Turn Signal/LConn1 -- Left Turn Signal/LConn1 -- Brake Lights/LConn1 -- BPS Run Light/LConn1 -- Headlights/LConn1
  - BPS Run Light/RConn1 -- BPS Run Light/LConn2
  - LTS/RConn1 -- Left Turn Signal/LConn2
  - Brake/RConn1 -- Brake Lights/LConn2
  - Headlights/RConn1 -- Headlights/LConn2

== system SolarCar/Dispersed/Steering Wheel ==
  12V : PMIOPort  Side=Right
  GND : PMIOPort  Port=2  Side=Right
  Essentials CANH : PMIOPort  Port=3  Side=Right
  Essentials CANL : PMIOPort  Port=4  Side=Right

== system SolarCar/Dispersed/Telemetry ==
  12V : PMIOPort  Side=Right
  GND : PMIOPort  Port=2  Side=Right
  Telemetry CANH : PMIOPort  Port=3  Side=Right
  Telemetry CANL : PMIOPort  Port=4  Side=Right

== system SolarCar/Dispersed/Throttle ==
  + Throttle Pot : PMIOPort  Side=Left
  - Throttle Pot : PMIOPort  Port=2  Side=Left
  Throttle Pot Signal : PMIOPort  Port=3  Side=Right

== system SolarCar/HV Box/100-12V ==
  + 100-12V In : PMIOPort  Side=Left
  - 100-12V In : PMIOPort  Port=2  Side=Left
  + 100-12V Out : PMIOPort  Port=3  Side=Right
  - 100-12V Out : PMIOPort  Port=4  Side=Right

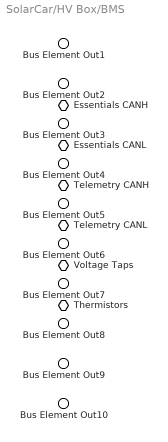
== system SolarCar/HV Box/BMS ==
  Essentials CANH : PMIOPort  Side=Left
  Essentials CANL : PMIOPort  Port=2  Side=Left
  Telemetry CANH : PMIOPort  Port=3  Side=Left
  Telemetry CANL : PMIOPort  Port=4  Side=Left
  Voltage Taps : PMIOPort  Port=5  Side=Left
  Thermistors : PMIOPort  Port=6  Side=Left
  Bus Element Out1 : Outport  PortName=+ Precharge Motor Coil
  Bus Element Out2 : Outport  Port=2  PortName=- Precharge Motor Coil
  Bus Element Out3 : Outport  Port=3  PortName=+ Motor Coil
  Bus Element Out4 : Outport  Port=4  PortName=- Motor Coil
  Bus Element Out5 : Outport  Port=5  PortName=+ Precharge MPPT Coil
  Bus Element Out6 : Outport  Port=6  PortName=- Precharge MPPT Coil
  Bus Element Out7 : Outport  Port=7  PortName=+ MPPT Coil
  Bus Element Out8 : Outport  Port=8  PortName=- MPPT Coil
  Bus Element Out9 : Outport  Port=9  PortName=+ Main Coil
  Bus Element Out10 : Outport  Port=10  PortName=- Main Coil

== system SolarCar/HV Box/Battery Pack ==
  Thermistors : PMIOPort  Side=Left
  Voltage Taps : PMIOPort  Port=2  Side=Left
  Bus Element Out2 : Outport  PortName=+
  Bus Element Out1 : Outport  Port=2  PortName=-

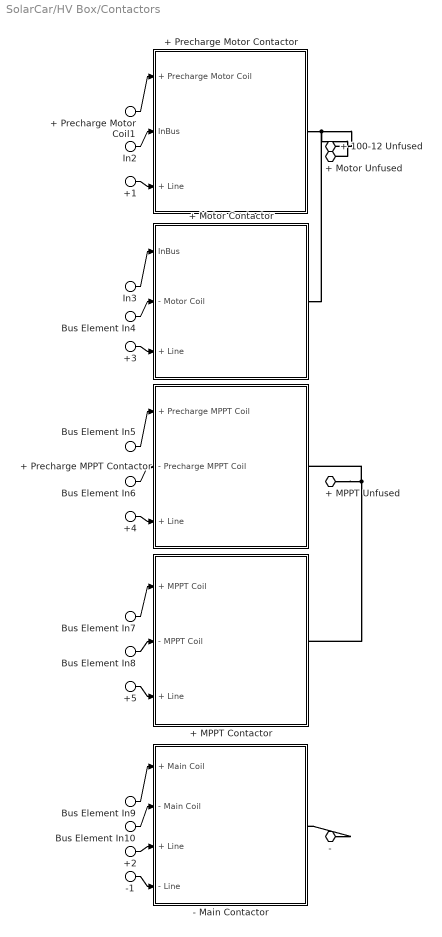
== system SolarCar/HV Box/Contactors ==
  + Precharge Motor Coil1 : Inport  PortName=+ Precharge Motor Coil
  In2 : Inport  Port=2  PortName=- Precharge Motor Coil
  In3 : Inport  Port=3  PortName=+ Motor Coil
  Bus Element In4 : Inport  Port=4  PortName=- Motor Coil
  Bus Element In5 : Inport  Port=5  PortName=+ Precharge MPPT Coil
  Bus Element In6 : Inport  Port=6  PortName=- Precharge MPPT Coil
  Bus Element In7 : Inport  Port=7  PortName=+ MPPT Coil
  Bus Element In8 : Inport  Port=8  PortName=- MPPT Coil
  Bus Element In9 : Inport  Port=9  PortName=+ Main Coil
  Bus Element In10 : Inport  Port=10  PortName=- Main Coil
  +{1..5} (5 alike) : Inport  Port=11  PortName=+ Line
  -1 : Inport  Port=12  PortName=- Line
  + MPPT Contactor : Subsystem
      settings: PortSchema="{\"entries\":[{\"content\":{\"headerSize\":26,\"margin\":15,\"minimumSpacing\":25,\"sides\":[{\"content\":{\"connectorIds\":[\"In1\",\"In2\",\"In3\"]},\"type\":\"ConnectorPlacement.EquallySpacedRectSide\",\"uuid\":\"c92e0290-dc73-43e5-9f21-68f158b061d1\"},{\"content\":{\"connectorIds\":[\"RConn1\"],\"side\":\"RIGHT\"},\"type\":\"ConnectorPlacement.EquallySpacedRectSide\",\"uuid\":\"be8eb41d-7a66-441b-b503-1306464e1273\"},{\"content\":{\"side\":\"TOP\"},\"type\":\"ConnectorPlacement.EquallySpacedRectSide\",\"uuid\":\"34016d46-a56f-490a-9c85-32531a59f6cc\"}]},\"type\":\"ConnectorPlacement.EquallySpacedConnector\",\"uuid\":\"21576b4b-d4ce-437a-96c9-76a257c64a5e\"}],\"packageUris\":[\"http://schema.mathworks.com/mf0/Connector/R2020b\"],\"version\":\"1.0\"}"
  + Motor Contactor : Subsystem
      settings: PortSchema="{\"entries\":[{\"content\":{\"headerSize\":26,\"margin\":15,\"minimumSpacing\":25,\"sides\":[{\"content\":{\"connectorIds\":[\"In1\",\"In2\",\"In3\"]},\"type\":\"ConnectorPlacement.EquallySpacedRectSide\",\"uuid\":\"c92e0290-dc73-43e5-9f21-68f158b061d1\"},{\"content\":{\"connectorIds\":[\"RConn1\"],\"side\":\"RIGHT\"},\"type\":\"ConnectorPlacement.EquallySpacedRectSide\",\"uuid\":\"be8eb41d-7a66-441b-b503-1306464e1273\"},{\"content\":{\"side\":\"TOP\"},\"type\":\"ConnectorPlacement.EquallySpacedRectSide\",\"uuid\":\"34016d46-a56f-490a-9c85-32531a59f6cc\"}]},\"type\":\"ConnectorPlacement.EquallySpacedConnector\",\"uuid\":\"21576b4b-d4ce-437a-96c9-76a257c64a5e\"}],\"packageUris\":[\"http://schema.mathworks.com/mf0/Connector/R2020b\"],\"version\":\"1.0\"}"
  + Precharge MPPT Contactor : Subsystem
      settings: PortSchema="{\"entries\":[{\"content\":{\"headerSize\":26,\"margin\":15,\"minimumSpacing\":25,\"sides\":[{\"content\":{\"connectorIds\":[\"In1\",\"In2\",\"In3\"]},\"type\":\"ConnectorPlacement.EquallySpacedRectSide\",\"uuid\":\"c92e0290-dc73-43e5-9f21-68f158b061d1\"},{\"content\":{\"connectorIds\":[\"RConn1\"],\"side\":\"RIGHT\"},\"type\":\"ConnectorPlacement.EquallySpacedRectSide\",\"uuid\":\"be8eb41d-7a66-441b-b503-1306464e1273\"},{\"content\":{\"side\":\"TOP\"},\"type\":\"ConnectorPlacement.EquallySpacedRectSide\",\"uuid\":\"34016d46-a56f-490a-9c85-32531a59f6cc\"}]},\"type\":\"ConnectorPlacement.EquallySpacedConnector\",\"uuid\":\"21576b4b-d4ce-437a-96c9-76a257c64a5e\"}],\"packageUris\":[\"http://schema.mathworks.com/mf0/Connector/R2020b\"],\"version\":\"1.0\"}"
  + Precharge Motor Contactor : Subsystem
      settings: PortSchema="{\"entries\":[{\"content\":{\"headerSize\":26,\"margin\":15,\"minimumSpacing\":25,\"sides\":[{\"content\":{\"connectorIds\":[\"In1\",\"In2\",\"In3\"]},\"type\":\"ConnectorPlacement.EquallySpacedRectSide\",\"uuid\":\"c92e0290-dc73-43e5-9f21-68f158b061d1\"},{\"content\":{\"connectorIds\":[\"RConn1\"],\"side\":\"RIGHT\"},\"type\":\"ConnectorPlacement.EquallySpacedRectSide\",\"uuid\":\"be8eb41d-7a66-441b-b503-1306464e1273\"},{\"content\":{\"side\":\"TOP\"},\"type\":\"ConnectorPlacement.EquallySpacedRectSide\",\"uuid\":\"34016d46-a56f-490a-9c85-32531a59f6cc\"}]},\"type\":\"ConnectorPlacement.EquallySpacedConnector\",\"uuid\":\"21576b4b-d4ce-437a-96c9-76a257c64a5e\"}],\"packageUris\":[\"http://schema.mathworks.com/mf0/Connector/R2020b\"],\"version\":\"1.0\"}"
  - Main Contactor : Subsystem
      settings: PortSchema="{\"entries\":[{\"content\":{\"headerSize\":26,\"margin\":15,\"minimumSpacing\":25,\"sides\":[{\"content\":{\"connectorIds\":[\"In1\",\"In2\",\"In3\",\"In4\"]},\"type\":\"ConnectorPlacement.EquallySpacedRectSide\",\"uuid\":\"c92e0290-dc73-43e5-9f21-68f158b061d1\"},{\"content\":{\"connectorIds\":[\"RConn1\"],\"side\":\"RIGHT\"},\"type\":\"ConnectorPlacement.EquallySpacedRectSide\",\"uuid\":\"be8eb41d-7a66-441b-b503-1306464e1273\"},{\"content\":{\"side\":\"TOP\"},\"type\":\"ConnectorPlacement.EquallySpacedRectSide\",\"uuid\":\"34016d46-a56f-490a-9c85-32531a59f6cc\"}]},\"type\":\"ConnectorPlacement.EquallySpacedConnector\",\"uuid\":\"21576b4b-d4ce-437a-96c9-76a257c64a5e\"}],\"packageUris\":[\"http://schema.mathworks.com/mf0/Connector/R2020b\"],\"version\":\"1.0\"}"
  + Motor Unfused : PMIOPort  Side=Right
  + MPPT Unfused : PMIOPort  Port=2  Side=Right
  + 100-12 Unfused : PMIOPort  Port=3  Side=Right
  - : PMIOPort  Port=4  Side=Right
  wires:
  -1/1 -> - Main Contactor/4(- Line)
  + Precharge Motor Coil1/1 -> + Precharge Motor Contactor/1(+ Precharge Motor Coil)
  In3/1 -> + Motor Contactor/1(InBus)
  In2/1 -> + Precharge Motor Contactor/2(InBus)
  Bus Element In4/1 -> + Motor Contactor/2(- Motor Coil)
  Bus Element In5/1 -> + Precharge MPPT Contactor/1(+ Precharge MPPT Coil)
  Bus Element In6/1 -> + Precharge MPPT Contactor/2(- Precharge MPPT Coil)
  Bus Element In7/1 -> + MPPT Contactor/1(+ MPPT Coil)
  Bus Element In8/1 -> + MPPT Contactor/2(- MPPT Coil)
  +2/1 -> - Main Contactor/3(+ Line)
  Bus Element In9/1 -> - Main Contactor/1(+ Main Coil)
  Bus Element In10/1 -> - Main Contactor/2(- Main Coil)
  +1/1 -> + Precharge Motor Contactor/3(+ Line)
  +3/1 -> + Motor Contactor/3(+ Line)
  +4/1 -> + Precharge MPPT Contactor/3(+ Line)
  +5/1 -> + MPPT Contactor/3(+ Line)
  connections:
  + Precharge Motor Contactor/RConn1 -- + Motor Unfused/RConn1 -- + 100-12 Unfused/RConn1 -- + Motor Contactor/RConn1
  + MPPT Unfused/RConn1 -- + MPPT Contactor/RConn1 -- + Precharge MPPT Contactor/RConn1
  -/RConn1 -- - Main Contactor/RConn1
